simulink model "H05_ARM"  (R2026a)
settings: Solver=VariableStepAuto  MaxStep=tau/25
InitFcn:
  | tau = 1;
libraries: MK_H x2
settings Model: Creator=Szalay  LastModifiedBy=Szalay

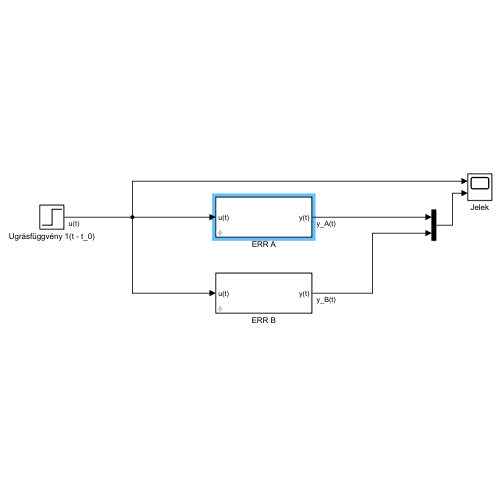
[thumbnail: Simulink's stored preview of the top-level diagram]
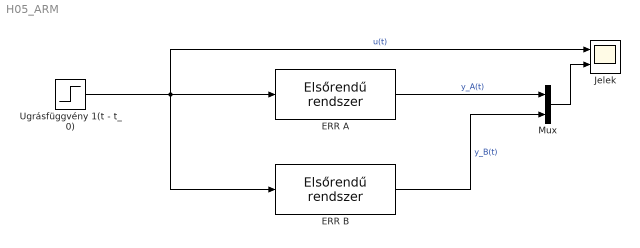
== system H05_ARM ==
  ERR A : MK_H/Elsőrendű rendszer  K=1  tau=tau  y_0=2.5
  ERR B : MK_H/Elsőrendű rendszer  K=1  tau=tau  y_0=2.5
  Jelek : Scope  NumInputPorts=2
      settings: ActiveDisplayYMinimum=-3.125  ActiveDisplayYMaximum=3.125
  Mux : Mux  Inputs=2
  Ugrásfüggvény 1(t - t_0) : Step  Time=5  FinalValue=0.5  SampleTime=0
  wires:
  Mux/1 -> Jelek/2
  Ugrásfüggvény 1(t - t_0)/1 -> ERR B/1, ERR A/1, Jelek/1  "u(t)"
  ERR A/1 -> Mux/1  "y_A(t)"
  ERR B/1 -> Mux/2  "y_B(t)"
